simulink model "lab09_nyquist_closed_loop_verification"  (R2025b)
settings: Solver=VariableStepAuto  StartTime=0.0  StopTime=10.0  RelTol=1e-3
settings Model: Creator=anshu  LastModifiedBy=anshu

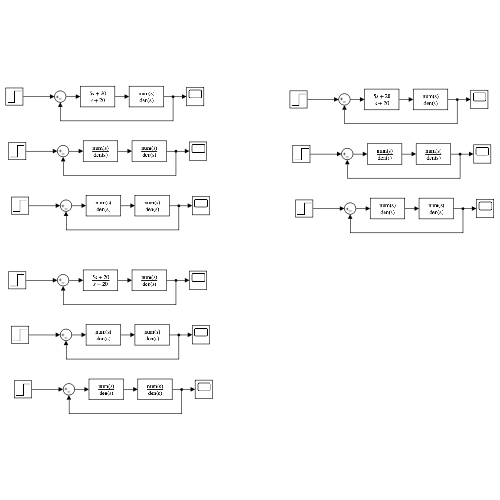
[thumbnail: Simulink's stored preview of the top-level diagram]
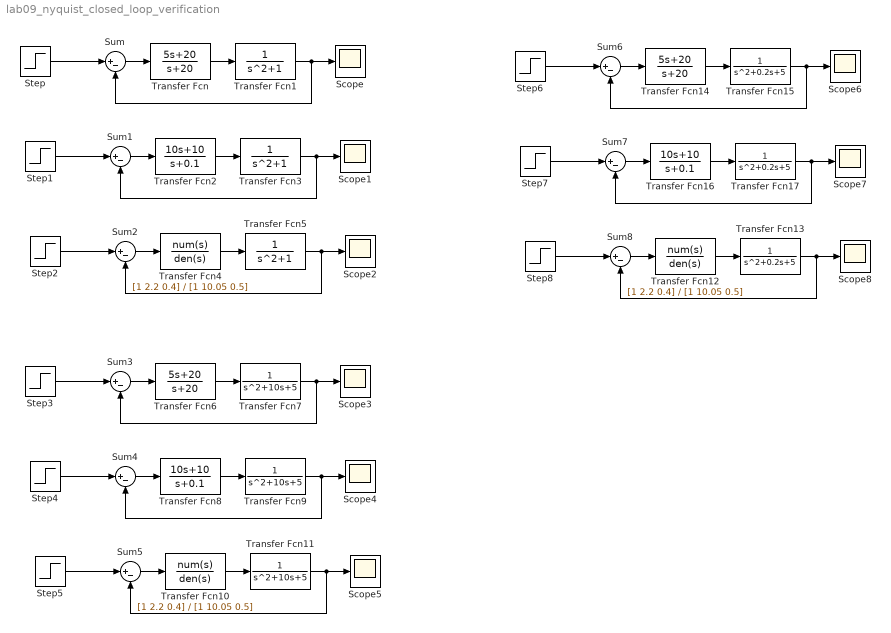
== system lab09_nyquist_closed_loop_verification ==
  Scope{,1..8} (9 alike) : Scope
      Scope settings: ActiveDisplayYMinimum=-1  ActiveDisplayYMaximum=1
      Scope1 settings: ActiveDisplayYMinimum=-1  ActiveDisplayYMaximum=1
      Scope2 settings: ActiveDisplayYMinimum=-1  ActiveDisplayYMaximum=1  DataLoggingVariableName=ScopeData2
      Scope3 settings: ActiveDisplayYMinimum=-1  ActiveDisplayYMaximum=1  DataLoggingVariableName=ScopeData3
      Scope4 settings: ActiveDisplayYMinimum=-0.12797393477252156  ActiveDisplayYMaximum=1.1517654129526942  DataLoggingVariableName=ScopeData4
      Scope5 settings: ActiveDisplayYMinimum=-0.0090309647152705431  ActiveDisplayYMaximum=0.0812786824374349  DataLoggingVariableName=ScopeData5
      Scope6 settings: ActiveDisplayYMinimum=-1  ActiveDisplayYMaximum=1  DataLoggingVariableName=ScopeData6
      Scope7 settings: ActiveDisplayYMinimum=-3.070258026233093  ActiveDisplayYMaximum=5.4229523142115479  DataLoggingVariableName=ScopeData7
      Scope8 settings: ActiveDisplayYMinimum=-0.011678454295722994  ActiveDisplayYMaximum=0.10510608866150696  DataLoggingVariableName=ScopeData8
  Step{,1..8} (9 alike) : Step  SampleTime=0
  Sum{,1..8} (9 alike) : Sum  Inputs=|+-
  Transfer Fcn : TransferFcn  Numerator=[5 20]  Denominator=[1 20]
  Transfer Fcn1 : TransferFcn  Denominator=[1 0 1]
  Transfer Fcn10 : TransferFcn  Numerator=[1 2.2 0.4]  Denominator=[1 10.05 0.5]
  Transfer Fcn11 : TransferFcn  Denominator=[1 10 5]
  Transfer Fcn12 : TransferFcn  Numerator=[1 2.2 0.4]  Denominator=[1 10.05 0.5]
  Transfer Fcn13 : TransferFcn  Denominator=[1 0.2 5]
  Transfer Fcn14 : TransferFcn  Numerator=[5 20]  Denominator=[1 20]
  Transfer Fcn15 : TransferFcn  Denominator=[1 0.2 5]
  Transfer Fcn16 : TransferFcn  Numerator=[10 10]  Denominator=[1 0.1]
  Transfer Fcn17 : TransferFcn  Denominator=[1 0.2 5]
  Transfer Fcn2 : TransferFcn  Numerator=[10 10]  Denominator=[1 0.1]
  Transfer Fcn3 : TransferFcn  Denominator=[1 0 1]
  Transfer Fcn4 : TransferFcn  Numerator=[1 2.2 0.4]  Denominator=[1 10.05 0.5]
  Transfer Fcn5 : TransferFcn  Denominator=[1 0 1]
  Transfer Fcn6 : TransferFcn  Numerator=[5 20]  Denominator=[1 20]
  Transfer Fcn7 : TransferFcn  Denominator=[1 10 5]
  Transfer Fcn8 : TransferFcn  Numerator=[10 10]  Denominator=[1 0.1]
  Transfer Fcn9 : TransferFcn  Denominator=[1 10 5]
  wires:
  Step/1 -> Sum/1
  Sum/1 -> Transfer Fcn/1
  Transfer Fcn1/1 -> Sum/2, Scope/1
  Transfer Fcn/1 -> Transfer Fcn1/1
  Transfer Fcn2/1 -> Transfer Fcn3/1
  Step1/1 -> Sum1/1
  Sum1/1 -> Transfer Fcn2/1
  Transfer Fcn3/1 -> Sum1/2, Scope1/1
  Transfer Fcn4/1 -> Transfer Fcn5/1
  Step2/1 -> Sum2/1
  Sum2/1 -> Transfer Fcn4/1
  Transfer Fcn5/1 -> Sum2/2, Scope2/1
  Transfer Fcn9/1 -> Sum4/2, Scope4/1
  Step4/1 -> Sum4/1
  Sum4/1 -> Transfer Fcn8/1
  Transfer Fcn8/1 -> Transfer Fcn9/1
  Transfer Fcn6/1 -> Transfer Fcn7/1
  Transfer Fcn7/1 -> Sum3/2, Scope3/1
  Step3/1 -> Sum3/1
  Transfer Fcn11/1 -> Sum5/2, Scope5/1
  Step5/1 -> Sum5/1
  Transfer Fcn10/1 -> Transfer Fcn11/1
  Sum3/1 -> Transfer Fcn6/1
  Sum5/1 -> Transfer Fcn10/1
  Transfer Fcn13/1 -> Sum8/2, Scope8/1
  Transfer Fcn12/1 -> Transfer Fcn13/1
  Transfer Fcn16/1 -> Transfer Fcn17/1
  Transfer Fcn17/1 -> Sum7/2, Scope7/1
  Sum8/1 -> Transfer Fcn12/1
  Step8/1 -> Sum8/1
  Step6/1 -> Sum6/1
  Transfer Fcn15/1 -> Sum6/2, Scope6/1
  Transfer Fcn14/1 -> Transfer Fcn15/1
  Sum7/1 -> Transfer Fcn16/1
  Step7/1 -> Sum7/1
  Sum6/1 -> Transfer Fcn14/1
